simulink model "DualBuckPPS22016_define"  (R2024b)
settings: Solver=ode45  StartTime=0.0  StopTime=0.5  RelTol=1e-3
model workspace (MAT data in the model file):
  D = 50
  T = 0.0333333333333
undefined symbols (not defined in the file): C, D_T_DOWN_Given, D_T_UP_Given, DiscIntNeverNeededParam, P, R, T_pulse, TP
libraries: spsOnDelayLib x27, dspsnks4 x12, dspfdesign x11, spsCurrentMeasurementLib x11, spsSeriesRLCBranchLib x8, spsMosfetLib x4, slpidlib x4, spsVoltageMeasurementLib x4, simulink x3, spsControlledCurrentSourceLib x1, spsDCVoltageSourceLib x1, spspowerguiLib x1
(part 2 of 2)

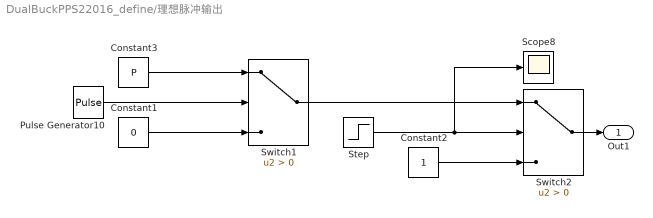
== system DualBuckPPS22016_define/理想脉冲输出 ==
  Constant1 : Constant  Value=0
  Constant2 : Constant
  Constant3 : Constant  Value=P
  Pulse Generator10 : DiscretePulseGenerator  PulseType=Time based  Period=T  PulseWidth=D  VectorParams1D=off
  Scope8 : Scope
  Step : Step  Time=0  SampleTime=0
  Switch1 : Switch  Criteria=u2 > Threshold  SaturateOnIntegerOverflow=off  InputSameDT=off
  Switch2 : Switch  Criteria=u2 > Threshold  SaturateOnIntegerOverflow=off  InputSameDT=off
  Out1 : Outport
  wires:
  Switch2/1 -> Out1/1
  Constant1/1 -> Switch1/3
  Step/1 -> Scope8/1, Switch2/2
  Switch1/1 -> Switch2/1
  Pulse Generator10/1 -> Switch1/2
  Constant2/1 -> Switch2/3
  Constant3/1 -> Switch1/1
